simulink model "InverterTest"  (R2026b)
settings: Solver=ode4  StopTime=fixtureCfg.Duration  FixedStep=experimentCfg.Step
PostLoadFcn:
  | addpath(fullfile(fileparts(fileparts(fileparts(fileparts(fileparts(get_param(bdroot,'FileName')))))),'docs','scripts'));initialize_motor_paths();initialize_motor_model(bdroot);
model workspace (MAT data in the model file):
  currentCfg.Ts = 0.0001
  currentCfg.BandwidthHz = 500
  currentCfg.Kpd = 3.14159265359
  currentCfg.Kpq = 3.76991118431
  currentCfg.Kid = 1570.79632679
  currentCfg.Kiq = 1570.79632679
  currentCfg.Kaw = 1000
  deadtimeCfg.DeadTime = 2e-06
  deadtimeCfg.DeviceDrop = 0
  deadtimeCfg.CurrentBlend = 0.1
  deadtimeCfg.ModelEnable = 0
  deadtimeCfg.CompensationEnable = 0
  deadtimeCfg.CompensationScale = 1
  deadtimeCfg.SwitchingStep = 1e-07
  experimentCfg.Step = 5e-06
  experimentCfg.LogTs = 0.0001
  experimentCfg.Duration = 1.5
  experimentCfg.Mode = 2
  experimentCfg.UseInverter = 1
  experimentCfg.UseTiming = 1
  experimentCfg.UseMechanical = 1
  experimentCfg.ImposedElectricalSpeed = 0
  experimentCfg.IdReference = 0
  experimentCfg.IqReference = 2
  experimentCfg.IqInitial = 0
  experimentCfg.SpeedReference = 40
  experimentCfg.SpeedInitial = 0
  experimentCfg.PositionReference = 1
  experimentCfg.PositionInitial = 0
  experimentCfg.CommandTime = 0.05
  experimentCfg.LoadTorque = 0.1
  experimentCfg.LoadTime = 0.35
  experimentCfg.Enable = 1
  experimentCfg.Reset = 0
  feedforwardCfg.Enable = 0
  feedforwardCfg.ParameterScale = 1
  fixtureCfg.Ts = 0.0001
  fixtureCfg.Duration = 0.03
  fixtureCfg.SolverStep = 5e-06
  fixtureCfg.VoltageAmplitude = 20
  fixtureCfg.FrequencyHz = 50
  fixtureCfg.InitialPhase = 0
  fixtureCfg.Inputs = [20 19.9901312073 19.9605345686 19.9112392921 19.8422940263 19.7537668119 19.6457450146 19.5183352388 19.3716632226 19.2058737135 19.0211303259 18.8176153791 ... (602 elements, 301x2)]
  inverterCfg.Vdc = 48
  inverterCfg.MinDuty = 0.02
  inverterCfg.PwmTs = 0.0001
  inverterCfg.LinearLimit = 26.6043004043
  motionCfg.Ts = 0.001
  motionCfg.NaturalFrequency = 20
  motionCfg.Damping = 0.9
  motionCfg.Kt = 0.21
  motionCfg.Kp = 0.0852380952381
  motionCfg.Ki = 0.952380952381
  motionCfg.Kaw = 20
  motionCfg.PositionKp = 8
  motionCfg.SpeedLimit = 80
  motionCfg.AccelerationLimit = 200
  motionCfg.CurrentLimit = 8
  pmsmCfg.Rs = 0.5
  pmsmCfg.Ld = 0.001
  pmsmCfg.Lq = 0.0012
  pmsmCfg.Flux = 0.035
  pmsmCfg.PolePairs = 4
  pmsmCfg.J = 0.0005
  pmsmCfg.B = 0.0001
  pmsmCfg.Id0 = 0
  pmsmCfg.Iq0 = 0
  pmsmCfg.Speed0 = 0
  pmsmCfg.Position0 = 0
  testStim.time = []
  testStim.signals.values = [20 19.9901312073 19.9605345686 19.9112392921 19.8422940263 19.7537668119 19.6457450146 19.5183352388 19.3716632226 19.2058737135 19.0211303259 18.8176153791 ... (602 elements, 301x2)]
  testStim.signals.dimensions = 2
  timingCfg.Ts = 0.0001
  timingCfg.FeedbackTicks = 1
  timingCfg.ActuationTicks = 1
libraries: Inverter x2, ClarkePark x1
settings Model: Creator=24322  LastModifiedBy=24322

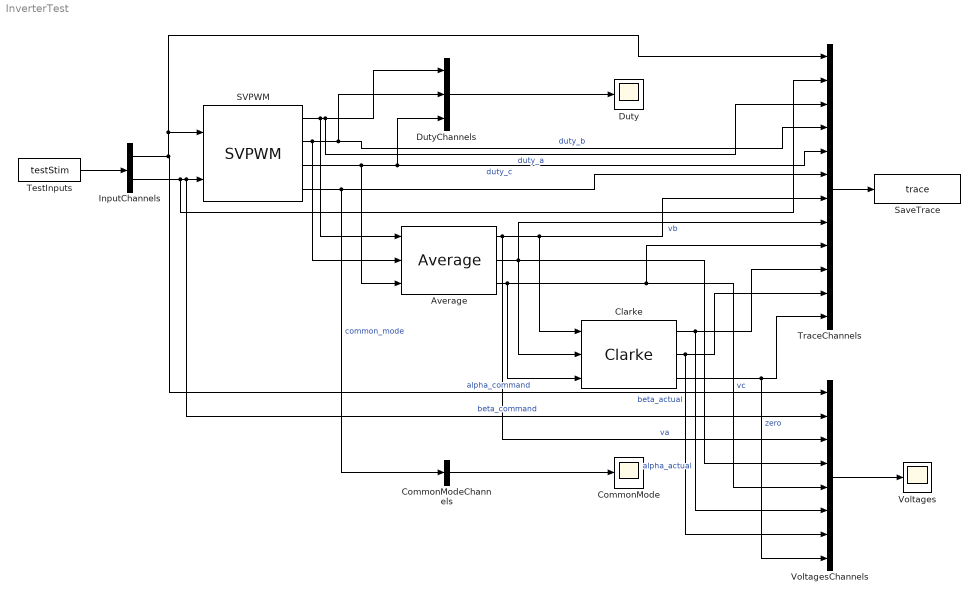
== system InverterTest ==
  Average : Inverter/Average  SystemSampleTime=-1  VariantActivationTime=update diagram  EmptyChoice=off  PassThrough=off  PassThroughVariantControl=(default)  EmptyChoiceVariantControl=(default)  AllowFlexibleInterface=on  Latency=0  AutoFrameSizeCalculation=off
  Clarke : ClarkePark/Clarke  SystemSampleTime=-1  VariantActivationTime=update diagram  EmptyChoice=off  PassThrough=off  PassThroughVariantControl=(default)  EmptyChoiceVariantControl=(default)  AllowFlexibleInterface=on  Latency=0  AutoFrameSizeCalculation=off
  CommonMode : Scope
      settings: Title=CommonMode  YLabel=V
  CommonModeChannels : Mux  Inputs=1
  Duty : Scope
      settings: Title=Duty  YLabel=1
  DutyChannels : Mux  Inputs=3
  InputChannels : Demux  Outputs=2
  SVPWM : Inverter/SVPWM  SystemSampleTime=-1  VariantActivationTime=update diagram  EmptyChoice=off  PassThrough=off  PassThroughVariantControl=(default)  EmptyChoiceVariantControl=(default)  AllowFlexibleInterface=on  Latency=0  AutoFrameSizeCalculation=off
  SaveTrace : ToWorkspace  VariableName=trace  SaveFormat=Structure With Time  SampleTime=experimentCfg.LogTs
  TestInputs : FromWorkspace  VariableName=testStim  SampleTime=currentCfg.Ts  Interpolate=off  OutputAfterFinalValue=Holding final value
  TraceChannels : Mux  Inputs=12
  Voltages : Scope
      settings: Title=Voltages  YLabel=V
  VoltagesChannels : Mux  Inputs=8
  wires:
  CommonModeChannels/1 -> CommonMode/1
  DutyChannels/1 -> Duty/1
  VoltagesChannels/1 -> Voltages/1
  Clarke/3 -> TraceChannels/12, VoltagesChannels/8  "zero"
  Clarke/2 -> TraceChannels/11, VoltagesChannels/7  "beta_actual"
  Clarke/1 -> TraceChannels/10, VoltagesChannels/6  "alpha_actual"
  SVPWM/4 -> TraceChannels/6, CommonModeChannels/1  "common_mode"
  TraceChannels/1 -> SaveTrace/1
  Average/3 -> TraceChannels/9, VoltagesChannels/5, Clarke/3  "vc"
  Average/2 -> Clarke/2, TraceChannels/8, VoltagesChannels/4  "vb"
  Average/1 -> Clarke/1, TraceChannels/7, VoltagesChannels/3  "va"
  SVPWM/3 -> DutyChannels/3, TraceChannels/5, Average/3  "duty_c"
  SVPWM/2 -> DutyChannels/2, TraceChannels/4, Average/2  "duty_b"
  SVPWM/1 -> TraceChannels/3, DutyChannels/1, Average/1  "duty_a"
  InputChannels/2 -> SVPWM/2, VoltagesChannels/2, TraceChannels/2  "beta_command"
  InputChannels/1 -> TraceChannels/1, SVPWM/1, VoltagesChannels/1  "alpha_command"
  TestInputs/1 -> InputChannels/1
